simulink model "one"  (R2026a)
settings: Solver=ode45  StopTime=tfin  RelTol=1e-6
values from neighbouring files (symbols this model uses):
  hdg0 = 0    [MATLAB_6b.m]    (also in lab6_c.m)
  L = 0.5    [MATLAB_6b.m]    (also in lab6_c.m)
  r = 0.1    [MATLAB_6b.m]    (also in lab6_c.m)
  x0 = 0    [MATLAB_6b.m]    (also in lab6_c.m)
  y0 = 0    [MATLAB_6b.m]    (also in lab6_c.m)
settings Model: Creator=m282256  LastModifiedBy=Owner

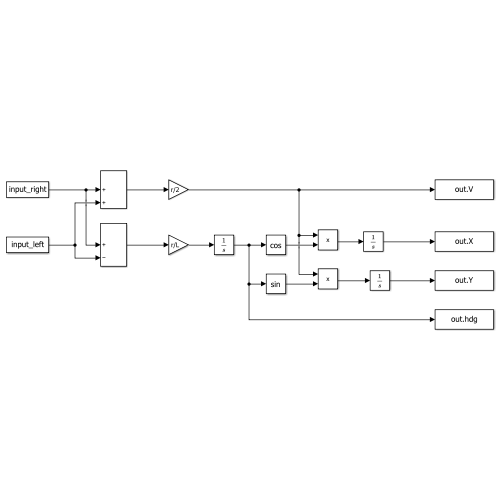
[thumbnail: Simulink's stored preview of the top-level diagram]
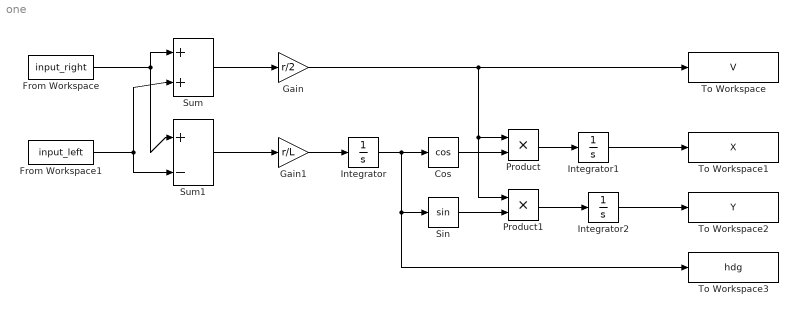
== system one ==
  Cos : Trigonometry  Operator=cos
  From Workspace : FromWorkspace  VariableName=input_right
  From Workspace1 : FromWorkspace  VariableName=input_left
  Gain : Gain  Gain=r/2
  Gain1 : Gain  Gain=r/L
  Integrator : Integrator  InitialCondition=hdg0
  Integrator1 : Integrator  InitialCondition=x0
  Integrator2 : Integrator  InitialCondition=y0
  Product : Product
  Product1 : Product
  Sin : Trigonometry
  Sum : Sum  Inputs=|++
  Sum1 : Sum  Inputs=|+-
  To Workspace : ToWorkspace  VariableName=V  SaveFormat=Timeseries  SampleTime=-1
  To Workspace1 : ToWorkspace  VariableName=X  SaveFormat=Timeseries  SampleTime=-1
  To Workspace2 : ToWorkspace  VariableName=Y  SaveFormat=Timeseries  SampleTime=-1
  To Workspace3 : ToWorkspace  VariableName=hdg  SaveFormat=Timeseries  SampleTime=-1
  wires:
  Sum1/1 -> Gain1/1
  Sum/1 -> Gain/1
  Gain1/1 -> Integrator/1
  Integrator/1 -> To Workspace3/1, Sin/1, Cos/1
  Cos/1 -> Product/2
  Product/1 -> Integrator1/1
  Sin/1 -> Product1/2
  Gain/1 -> Product1/1, Product/1, To Workspace/1
  Integrator1/1 -> To Workspace1/1
  Integrator2/1 -> To Workspace2/1
  Product1/1 -> Integrator2/1
  From Workspace/1 -> Sum1/1, Sum/1
  From Workspace1/1 -> Sum1/2, Sum/2
